simulink model "INS"  (R2018b)
settings: configuration reference "ins_config" (kept outside this file)
values from neighbouring files (symbols this model uses):
  INS_EXPORT = Simulink.Parameter(INS_EXPORT_VALUE)    [ins_model_init.m]
  INS_PARAM = Simulink.Parameter(INS_PARAM_VALUE)    [ins_model_init.m]
undefined symbols (not defined in the file or in its folder): DiscIntNeverNeededParam, INS_CONST, INS_EXPORT_VALUE, Sensor_Meas
libraries: simulink x131, FMT_Model_Lib x48
(part 6 of 6)

== system INS/Data_Fusion/Translation_Filter/CF/Verticle_Filter/Correct/ExternalPos_Correct/ExternalPos_Correct/Measurement/Bias_Estimation ==
  h_m : Inport
  TF_Data : Inport  Port=2
  X : Inport  Port=3
  Bias : Subsystem
  Bus Selector1 : BusSelector  OutputSignals=Sensor_Enable.vert_select.extpos_enable
  Delay : Delay  DelayLength=1
  Detect Increase : simulink/Logic and Bit Operations/Detect Increase  vinit=0  OutDataTypeStr=boolean
  Selector : Selector  InputPortWidth=3  IndexOptions=Index vector (dialog)  Indices=1  OutputSizes=1
  Switch : Switch  Criteria=u2 > Threshold  OutDataTypeStr=single
  bias : Outport
  bias_update : Outport  Port=2
  wires:
  Delay/1 -> Switch/3
  X/1 -> Selector/1
  Bias/1(bias) -> Switch/1
  Switch/1 -> Delay/1, bias/1  "extpos_alt_bias"
  Selector/1 -> Bias/1(height_est_m)
  h_m/1 -> Bias/2(height_meas_m)
  Bus Selector1/1 -> Detect Increase/1  "<extpos_enable>"
  TF_Data/1 -> Bus Selector1/1
  Detect Increase/1 -> bias_update/1, Switch/2  "extpos_bias_update"

== system INS/Data_Fusion/Translation_Filter/CF/Verticle_Filter/Correct/GPS_Correct/GPS_Correct/Error_Scaling/GPS_Error_Scaling ==
  error_in : Inport
  Demux : Demux  Outputs=2
  Gain : Gain  Gain=INS_PARAM.GPS_VEL_GAIN  OutDataTypeStr=single
  Gain1 : Gain  Gain=INS_PARAM.GPS_ALT_GAIN  OutDataTypeStr=single
  Gain2 : Gain  Gain=-INS_PARAM.GPS_BIAS_A_GAIN  OutDataTypeStr=single
  Gain4 : Gain  Gain=-0.75
  Mux : Mux  Inputs=3
  Sum : Sum  Inputs=++|
  error_out : Outport
  wires:
  Gain1/1 -> Gain4/1, Mux/1
  Gain2/1 -> Mux/3
  error_in/1 -> Demux/1
  Sum/1 -> Mux/2
  Demux/1 -> Gain1/1
  Demux/2 -> Gain2/1, Gain/1
  Gain4/1 -> Sum/1
  Gain/1 -> Sum/2
  Mux/1 -> error_out/1

== system INS/Data_Fusion/Translation_Filter/CF/Verticle_Filter/Correct/GPS_Correct/GPS_Correct/Error_Scaling/RTK_Error_Scaling ==
  error_in : Inport
  Demux : Demux  Outputs=2
  Gain : Gain  Gain=INS_PARAM.RTK_VEL_GAIN  OutDataTypeStr=single
  Gain1 : Gain  Gain=INS_PARAM.RTK_ALT_GAIN  OutDataTypeStr=single
  Gain2 : Gain  Gain=-INS_PARAM.RTK_BIAS_A_GAIN  OutDataTypeStr=single
  Gain4 : Gain  Gain=-0.75
  Mux : Mux  Inputs=3
  Sum : Sum  Inputs=++|
  error_out : Outport
  wires:
  Mux/1 -> error_out/1
  Gain/1 -> Sum/2
  Gain4/1 -> Sum/1
  Demux/2 -> Gain/1, Gain2/1
  Demux/1 -> Gain1/1
  Sum/1 -> Mux/2
  error_in/1 -> Demux/1
  Gain2/1 -> Mux/3
  Gain1/1 -> Mux/1, Gain4/1

== system INS/Data_Fusion/Translation_Filter/CF/Verticle_Filter/Correct/GPS_Correct/GPS_Correct/Measurement/Bias_Estimation ==
  h_m : Inport
  X : Inport  Port=2
  TF_Data : Inport  Port=3
  Bias : Subsystem
  Bus Selector1 : BusSelector  OutputSignals=Sensor_Enable.vert_select.gps_enable,Sensor_Status.GPS_Status.rtk_valid
  Detect Change : simulink/Logic and Bit Operations/Detect Change  vinit=0  OutDataTypeStr=boolean
  Detect Increase : simulink/Logic and Bit Operations/Detect Increase  vinit=0.0  OutDataTypeStr=boolean
  Logical Operator : Logic  Operator=OR  AllPortsSameDT=off  OutDataTypeStr=boolean
  Memory : Memory
  Selector : Selector  InputPortWidth=3  IndexOptions=Index vector (dialog)  Indices=1  OutputSizes=1
  Switch : Switch  Criteria=u2 > Threshold  OutDataTypeStr=single
  bias : Outport
  bias_update : Outport  Port=2
  wires:
  Memory/1 -> Switch/3
  X/1 -> Selector/1
  Bias/1(bias) -> Switch/1
  Switch/1 -> Memory/1, bias/1  "gps_height_bias"
  Selector/1 -> Bias/1(h_est_m)  "h_est_m1"
  Bus Selector1/1 -> Detect Increase/1  "<gps_enable>"
  Logical Operator/1 -> bias_update/1, Switch/2
  TF_Data/1 -> Bus Selector1/1
  h_m/1 -> Bias/2(h_meas_m)  "gps_h_meas"
  Bus Selector1/2 -> Detect Change/1  "<rtk_valid>"
  Detect Increase/1 -> Logical Operator/1
  Detect Change/1 -> Logical Operator/2

== system INS/Data_Fusion/Translation_Filter/CF/Verticle_Filter/Correct/Rf_Correct/Rangefinder_Correct/Measurement/Bias_Estimation ==
  h_m : Inport
  X : Inport  Port=2
  TF_Data : Inport  Port=3
  Bias : Subsystem
  Bus Selector1 : BusSelector  OutputSignals=Sensor_Enable.vert_select.rf_enable
  Bus Selector2 : BusSelector  OutputSignals=Sensor_Meas.Rf_Meas.timestamp_ms
  Detect Increase : simulink/Logic and Bit Operations/Detect Increase  vinit=0.0  OutDataTypeStr=boolean
  Detect_Jump_Signal : Subsystem
  Logical Operator : Logic  Operator=OR  AllPortsSameDT=off  OutDataTypeStr=boolean
  Memory : Memory
  Selector : Selector  InputPortWidth=3  IndexOptions=Index vector (dialog)  Indices=1  OutputSizes=1
  Switch : Switch  Criteria=u2 > Threshold  OutDataTypeStr=single
  bias : Outport
  bias_update : Outport  Port=2
  wires:
  Memory/1 -> Switch/3
  X/1 -> Selector/1
  Bias/1(bias) -> Switch/1
  Switch/1 -> Memory/1, bias/1  "rf_height_bias"
  Selector/1 -> Bias/1(h_est_m)  "rf_h_est_m"
  Bus Selector1/1 -> Detect Increase/1  "<rf_enable>"
  Logical Operator/1 -> bias_update/1, Switch/2
  TF_Data/1 -> Bus Selector2/1, Bus Selector1/1
  h_m/1 -> Detect_Jump_Signal/1(h_meas_m), Bias/2(h_meas_m)  "rf_h_meas"
  Bus Selector2/1 -> Detect_Jump_Signal/2(timestamp)  "<timestamp_ms>"
  Detect Increase/1 -> Logical Operator/1
  Detect_Jump_Signal/1(update) -> Logical Operator/2

== system INS/Data_Fusion/Translation_Filter/CF/Verticle_Filter/Predict/Propagate/States_Init/Height_Init/Baro_Reference_Height ==
  TF_Data : Inport
  Enable : EnablePort
  Bus Selector : BusSelector  OutputSignals=Sensor_Meas.Baro_Meas.h_R_m
  Data Type Conversion : DataTypeConversion  OutDataTypeStr=single
  h_R_m : Outport
  wires:
  Data Type Conversion/1 -> h_R_m/1
  Bus Selector/1 -> Data Type Conversion/1  "<h_R_m>"
  TF_Data/1 -> Bus Selector/1

== system INS/Data_Fusion/Translation_Filter/CF/Verticle_Filter/Predict/Propagate/States_Init/Height_Init/External_Pos_Height ==
  TF_Data : Inport
  Enable : EnablePort
  Bus Selector : BusSelector  OutputSignals=Sensor_Meas.ExtPos_Meas.h_O_m
  Data Type Conversion : DataTypeConversion  OutDataTypeStr=single
  h_R_m : Outport
  wires:
  TF_Data/1 -> Bus Selector/1
  Bus Selector/1 -> Data Type Conversion/1  "<h_O_m>"
  Data Type Conversion/1 -> h_R_m/1

== system INS/Data_Fusion/Translation_Filter/CF/Verticle_Filter/Predict/Propagate/States_Init/Height_Init/GPS_Reference_Height ==
  TF_Data : Inport
  Enable : EnablePort
  Bus Selector : BusSelector  OutputSignals=Sensor_Meas.GPS_Meas.h_m
  Data Type Conversion : DataTypeConversion  OutDataTypeStr=single
  h_R_m : Outport
  wires:
  Data Type Conversion/1 -> h_R_m/1
  Bus Selector/1 -> Data Type Conversion/1  "<h_m>"
  TF_Data/1 -> Bus Selector/1

== system INS/Data_Fusion/Translation_Filter/CF/Verticle_Filter/Predict/Propagate/States_Init/Height_Init/Rf_Reference_Height ==
  TF_Data : Inport
  Enable : EnablePort
  Bus Selector : BusSelector  OutputSignals=Sensor_Meas.Rf_Meas.h_AGL_m
  Data Type Conversion : DataTypeConversion  OutDataTypeStr=single
  h_R_m : Outport
  wires:
  TF_Data/1 -> Bus Selector/1
  Bus Selector/1 -> Data Type Conversion/1  "<h_AGL_m>"
  Data Type Conversion/1 -> h_R_m/1

== system INS/Data_Fusion/Translation_Filter/CF/Verticle_Filter/Predict/Propagate/States_Init/Velocity_Init/Baro_Velocity ==
  TF_Data : Inport
  Enable : EnablePort
  Constant : Constant  Value=0  OutDataTypeStr=single
  Terminator : Terminator
  vel_D_mPs : Outport
  wires:
  Constant/1 -> vel_D_mPs/1
  TF_Data/1 -> Terminator/1

== system INS/Data_Fusion/Translation_Filter/CF/Verticle_Filter/Predict/Propagate/States_Init/Velocity_Init/GPS_Velocity ==
  TF_Data : Inport
  Enable : EnablePort
  Bus Selector : BusSelector  OutputSignals=Sensor_Meas.GPS_Meas.vd_mPs
  Data Type Conversion : DataTypeConversion  OutDataTypeStr=single
  vel_D_mPs : Outport
  wires:
  Data Type Conversion/1 -> vel_D_mPs/1
  Bus Selector/1 -> Data Type Conversion/1  "<vd_mPs>"
  TF_Data/1 -> Bus Selector/1

== system INS/Data_Fusion/Translation_Filter/CF/Verticle_Filter/Predict/Propagate/States_Init/Velocity_Init/Rf_Velocity ==
  TF_Data : Inport
  Enable : EnablePort
  Constant : Constant  Value=0  OutDataTypeStr=single
  Terminator : Terminator
  vel_D_mPs : Outport
  wires:
  Constant/1 -> vel_D_mPs/1
  TF_Data/1 -> Terminator/1

== system INS/Data_Fusion/Translation_Filter/CF/Horizontal_Filter/Correct/ExternalPos Correct/ExternalPos_Correct/Measurement/Bias_Estimation/Bias ==
  xy_est_m : Inport
  xy_meas_m : Inport  Port=2
  Sum : Sum  Inputs=+-|
  bias : Outport
  wires:
  Sum/1 -> bias/1
  xy_meas_m/1 -> Sum/2  "xy_meas_m"
  xy_est_m/1 -> Sum/1  "xy_est_m"

== system INS/Data_Fusion/Translation_Filter/CF/Horizontal_Filter/Correct/GPS Correct/GPS_Correct/Measurement/Bias_Estimation/Bias ==
  xy_meas_m : Inport
  X : Inport  Port=2
  TF_Data : Inport  Port=3
  Bias_Update : Subsystem
  Bus Selector1 : BusSelector  OutputSignals=Sensor_Status.GPS_Status.rtk_valid,Sensor_Enable.horizon_select.gps_enable
  Detect Change : simulink/Logic and Bit Operations/Detect Change  vinit=0  OutDataTypeStr=boolean
  Detect Increase : simulink/Logic and Bit Operations/Detect Increase  vinit=0.0  OutDataTypeStr=boolean
  Logical Operator : Logic  Operator=OR  AllPortsSameDT=off  OutDataTypeStr=boolean
  Memory : Memory  InitialCondition=[0;0]
  Selector : Selector  InputPortWidth=7  IndexOptions=Index vector (dialog)  Indices=[1 2]  OutputSizes=1
  Switch : Switch  Criteria=u2 > Threshold  OutDataTypeStr=single
  bias : Outport
  bias_update : Outport  Port=2
  wires:
  xy_meas_m/1 -> Bias_Update/2(xy_meas_m)
  TF_Data/1 -> Bias_Update/3(TF_Data), Bus Selector1/1
  Logical Operator/1 -> bias_update/1, Switch/2
  Bus Selector1/2 -> Detect Increase/1  "<gps_enable>"
  Selector/1 -> Bias_Update/1(xy_est_m)  "gps_xy_est"
  Switch/1 -> bias/1, Memory/1  "gps_pos_bias"
  Bias_Update/1(bias) -> Switch/1
  X/1 -> Selector/1
  Memory/1 -> Switch/3
  Bus Selector1/1 -> Detect Change/1  "<rtk_valid>"
  Detect Change/1 -> Logical Operator/1
  Detect Increase/1 -> Logical Operator/2

== system INS/Data_Fusion/Translation_Filter/CF/Verticle_Filter/Correct/Baro_Correct/Baro_Correct/Measurement/Bias_Estimation/Bias ==
  height_est_m : Inport
  height_meas_m : Inport  Port=2
  Sum : Sum  Inputs=+-|
  bias : Outport
  wires:
  Sum/1 -> bias/1
  height_meas_m/1 -> Sum/2  "height_meas_m"
  height_est_m/1 -> Sum/1  "height_est_m"

== system INS/Data_Fusion/Translation_Filter/CF/Verticle_Filter/Correct/ExternalPos_Correct/ExternalPos_Correct/Measurement/Bias_Estimation/Bias ==
  height_est_m : Inport
  height_meas_m : Inport  Port=2
  Sum : Sum  Inputs=+-|
  bias : Outport
  wires:
  Sum/1 -> bias/1
  height_meas_m/1 -> Sum/2  "height_meas_m"
  height_est_m/1 -> Sum/1  "height_est_m"

== system INS/Data_Fusion/Translation_Filter/CF/Verticle_Filter/Correct/GPS_Correct/GPS_Correct/Measurement/Bias_Estimation/Bias ==
  h_est_m : Inport
  h_meas_m : Inport  Port=2
  Sum : Sum  Inputs=+-|
  bias : Outport
  wires:
  h_meas_m/1 -> Sum/2
  h_est_m/1 -> Sum/1
  Sum/1 -> bias/1

== system INS/Data_Fusion/Translation_Filter/CF/Verticle_Filter/Correct/Rf_Correct/Rangefinder_Correct/Measurement/Bias_Estimation/Bias ==
  h_est_m : Inport
  h_meas_m : Inport  Port=2
  Sum : Sum  Inputs=+-|
  bias : Outport
  wires:
  Sum/1 -> bias/1
  h_meas_m/1 -> Sum/2
  h_est_m/1 -> Sum/1

== system INS/Data_Fusion/Translation_Filter/CF/Verticle_Filter/Correct/Rf_Correct/Rangefinder_Correct/Measurement/Bias_Estimation/Detect_Jump_Signal ==
  h_meas_m : Inport
  timestamp : Inport  Port=2
  Abs : Abs
  Compare To Constant : simulink/Logic and Bit Operations/Compare To Constant  relop=>  const=5  OutDataTypeStr=boolean
  Constant : Constant  Value=100  OutDataTypeStr=uint32
  Constant1 : Constant  Value=1000  OutDataTypeStr=single
  Delay : Delay  DelayLength=1
  Delay1 : Delay  DelayLength=1  InitialConditionSource=Input port
      settings: InputPortMap=u0,p4
  Delay2 : Delay  DelayLength=1  InitialCondition=0
  Detect Increase : simulink/Logic and Bit Operations/Detect Increase  vinit=0.0  OutDataTypeStr=boolean
  Divide : Product  Inputs=*/
  Multiply : Product
  Sum : Sum  Inputs=|+-
  Sum1 : Sum  Inputs=|+-
  Switch : Switch  Criteria=u2 > Threshold
  Switch1 : Switch  Criteria=u2 > Threshold
  update : Outport
  wires:
  h_meas_m/1 -> Sum/1, Delay/1
  Delay/1 -> Sum/2
  Sum/1 -> Multiply/1
  Multiply/1 -> Abs/1
  Abs/1 -> Compare To Constant/1  "rf_jump"
  timestamp/1 -> Sum1/1, Detect Increase/1, Delay1/2, Delay1/1
  Detect Increase/1 -> Switch/2
  Switch/1 -> Delay2/1, Switch1/1, Switch1/2  "timespan"
  Delay2/1 -> Switch/3
  Sum1/1 -> Switch/1
  Delay1/1 -> Sum1/2
  Constant/1 -> Switch1/3
  Switch1/1 -> Divide/2
  Constant1/1 -> Divide/1
  Divide/1 -> Multiply/2  "1/dT"
  Compare To Constant/1 -> update/1

== system INS/Data_Fusion/Translation_Filter/CF/Horizontal_Filter/Correct/GPS Correct/GPS_Correct/Measurement/Bias_Estimation/Bias/Bias_Update ==
  note: If RTK is valid and onground, then we
      | position converge to RTK position
  xy_est_m : Inport
  xy_meas_m : Inport  Port=2
  TF_Data : Inport  Port=3
  Bus Selector : BusSelector  OutputSignals=Sensor_Status.GPS_Status.rtk_valid,Sensor_Status.GPS_Status.standstill
  Constant : Constant  Value=0  OutDataTypeStr=single
  Logical Operator : Logic  AllPortsSameDT=off  OutDataTypeStr=boolean
  Sum : Sum  Inputs=+-|
  Switch : Switch  Criteria=u2 > Threshold
  bias : Outport
  wires:
  xy_est_m/1 -> Sum/1
  xy_meas_m/1 -> Sum/2
  TF_Data/1 -> Bus Selector/1
  Bus Selector/1 -> Logical Operator/1  "<rtk_valid>"
  Logical Operator/1 -> Switch/2
  Switch/1 -> bias/1
  Sum/1 -> Switch/3
  Constant/1 -> Switch/1
  Bus Selector/2 -> Logical Operator/2  "<standstill>"

== matlab function INS/Sensor_PreProcess/GPS_PreProcess/Data_Scalling/saturation/Rem ==
  data: a input; y output; b input
function y = fcn(a, b)

y = a - b.*fix(a./b);
